simulink model "VHDModel"  (R2021b)
settings: Solver=VariableStepAuto  StartTime=0.0  StopTime=30  RelTol=1e-3
values from neighbouring files (symbols this model uses):
  CG_TO_FRONT_AXLE = 1.56    [VHD_parameters.m]
  CG_TO_REAR_AXLE = 1.04    [VHD_parameters.m]
  COEFICEINT_OF_FRICTION = 0.8    [VHD_parameters.m]
  FRONT_LATERAL_COEF = 14    [VHD_parameters.m]
  INERTIAL_MASS_MOMENT = 1360    [VHD_parameters.m]
  REAR_LATERAL_COEF = 13    [VHD_parameters.m]
  STEERING_RATIO = 1    [VHD_parameters.m]
  VEHICLE_MASS = 1600    [VHD_parameters.m]
  VEHICLE_TRACK = 1.7    [VHD_parameters.m]
  VELOCITY = 40    [VHD_parameters.m]
  WHEEL_BASE = 2.6    [VHD_parameters.m]
undefined symbols (not defined in the file or in its folder): magnitude
libraries: slpidlib x2, simulink_extras x2, simulink x1

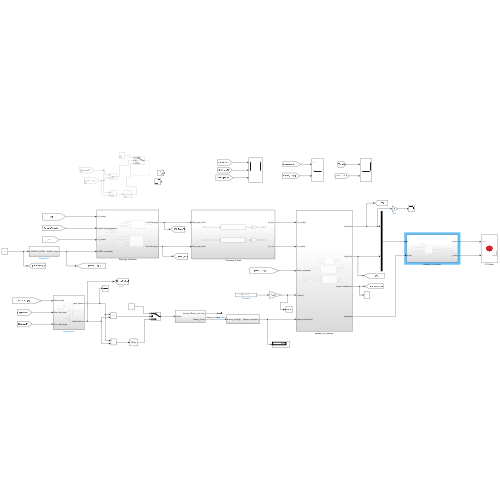
[thumbnail: Simulink's stored preview of the top-level diagram]
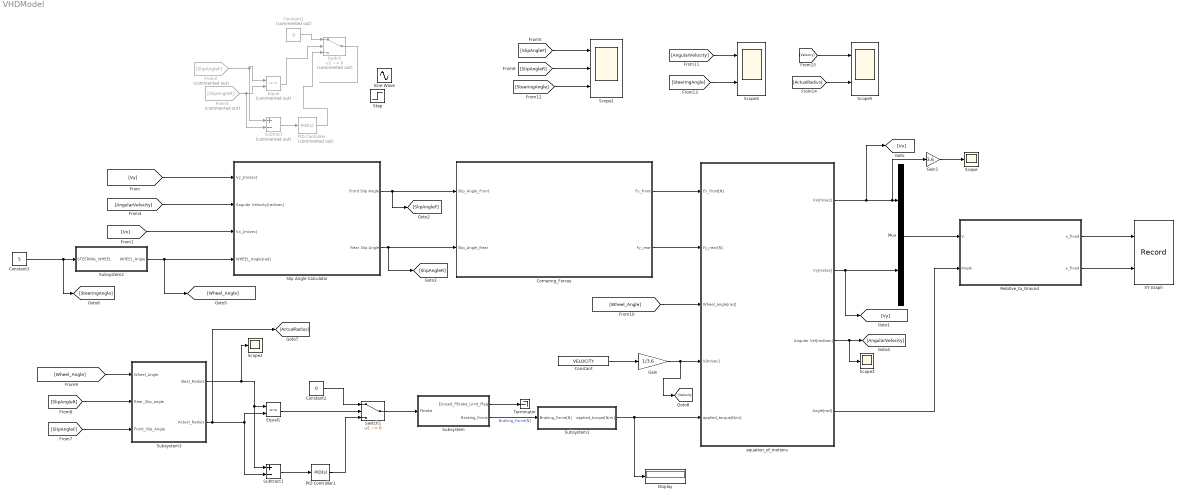
== system VHDModel ==
  Constant : Constant  Value=VELOCITY
  Constant1 : Constant  Commented=on  Value=0
  Constant2 : Constant  Value=0
  Constant3 : Constant  Value=5
  Cornering_Forces : Subsystem
  Display : Display
  Equal : RelationalOperator  Commented=on  Operator===  OutDataTypeStr=boolean  RndMeth=Simplest
  Equal1 : RelationalOperator  Operator===  OutDataTypeStr=boolean  RndMeth=Simplest
  From2 : From  Commented=on  GotoTag=SlipAngleF
  From3 : From  Commented=on  GotoTag=SlipAngleR
  Gain : Gain  Gain=1/3.6
  Gain1 : Gain  Gain=3.6
  Mux : Mux  Inputs=2
  PID Controller : slpidlib/PID Controller  Commented=on  Controller=PID  Form=Parallel  TimeDomain=Continuous-time  UseExternalTs=off  SampleTime=-1  IntegratorMethod=Forward Euler  FilterMethod=Forward Euler  ControllerParametersSource=internal  P=82.330505190178  I=12407.3336326962  D=0.077849176466117  UseFilter=on  N=20851.8597553552  TunerSelectOption=Transfer Function Based (PID Tuner App)  InitialConditionSource=internal  InitialConditionForIntegrator=0  InitialConditionForFilter=0  DifferentiatorICPrevScaledInput=0  ExternalReset=none  TrackingMode=off  Kt=1  LimitOutput=off  SatLimitsSource=internal  UpperSaturationLimit=inf  LowerSaturationLimit=-inf  LinearizeAsGain=on  AntiWindupMode=none  Kb=1  POutMin=[]  POutMax=[]  IOutMin=[]  IOutMax=[]  DOutMin=[]  DOutMax=[]  NOutMin=[]  NOutMax=[]  SumOutMin=[]  SumOutMax=[]  SaturationOutMin=[]  SaturationOutMax=[]  PParamMin=[]  PParamMax=[]  IParamMin=[]  IParamMax=[]  DParamMin=[]  DParamMax=[]  NParamMin=[]  NParamMax=[]  KbParamMin=[]  KbParamMax=[]  KtParamMin=[]  KtParamMax=[]  KbOutMin=[]  KbOutMax=[]  KtOutMin=[]  KtOutMax=[]  IntegratorOutMin=[]  IntegratorOutMax=[]  FilterOutMin=[]  FilterOutMax=[]  SumI1OutMin=[]  SumI1OutMax=[]  SumI2OutMin=[]  SumI2OutMax=[]  SumI3OutMin=[]  SumI3OutMax=[]  SumI4OutMin=[]  SumI4OutMax=[]  SumDOutMin=[]  SumDOutMax=[]  DifferentiatorOutMin=[]  DifferentiatorOutMax=[]  FilterDiffOutCoefMin=[]  FilterDiffOutCoefMax=[]  ReciprocalOutMin=[]  ReciprocalOutMax=[]  SumDenOutMin=[]  SumDenOutMax=[]  SumNumOutMin=[]  SumNumOutMax=[]  DivideOutMin=[]  DivideOutMax=[]  UdiffTsProdOutMin=[]  UdiffTsProdOutMax=[]  NTsProdOutMin=[]  NTsProdOutMax=[]  UintegralTsProdOutMin=[]  UintegralTsProdOutMax=[]  UngainTsProdOutMin=[]  UngainTsProdOutMax=[]  IntegratorContinuousStateAttributes=''  IntegratorStateMustResolveToSignalObject=off  IntegratorRTWStateStorageClass=Auto  FilterContinuousStateAttributes=''  FilterStateMustResolveToSignalObject=off  FilterRTWStateStorageClass=Auto  ParallelPVariant=InternalParameters  IdealPVariant=Disabled  IVariant=InternalParameters  DVariant=InternalParameters  IntegratorVariant=Continuous  SatVariant=Disabled  AWVariant=Passthrough  PCopyVariant=Disabled  TRVariant=Disabled  FdbkBlocksVariant=Forward  IdealPFdbkVariant=Disabled  SatFdbkVariant=Disabled  DerivativeFilterVariant=ContFilter  NVariant=InternalParameters  NCopyVariant=Disabled  FilterICVariant=InternalICsFilter  IntegratorICVariant=InternalICs  ExternalResetVariant=Disabled  TRSumVariant=Passthrough  SumFdbkVariant=Disabled  SumVariant=Sum_PID  TsampFilterVariant=InternalTs  TsampNgainVariant=Passthrough  TsampIntegralVariant=Passthrough  ExternalSaturationOutDataTypeStr=Inherit: Same as second input
  PID Controller1 : slpidlib/PID Controller  Controller=PID  Form=Parallel  TimeDomain=Continuous-time  UseExternalTs=off  SampleTime=-1  IntegratorMethod=Forward Euler  FilterMethod=Forward Euler  ControllerParametersSource=internal  P=-765.564265691975  I=-781534.171021295  D=-0.0269112999506061  UseFilter=on  N=5836.60149931409  TunerSelectOption=Transfer Function Based (PID Tuner App)  InitialConditionSource=internal  InitialConditionForIntegrator=0  InitialConditionForFilter=0  DifferentiatorICPrevScaledInput=0  ExternalReset=none  TrackingMode=off  Kt=1  LimitOutput=off  SatLimitsSource=internal  UpperSaturationLimit=inf  LowerSaturationLimit=-inf  LinearizeAsGain=on  AntiWindupMode=none  Kb=1  POutMin=[]  POutMax=[]  IOutMin=[]  IOutMax=[]  DOutMin=[]  DOutMax=[]  NOutMin=[]  NOutMax=[]  SumOutMin=[]  SumOutMax=[]  SaturationOutMin=[]  SaturationOutMax=[]  PParamMin=[]  PParamMax=[]  IParamMin=[]  IParamMax=[]  DParamMin=[]  DParamMax=[]  NParamMin=[]  NParamMax=[]  KbParamMin=[]  KbParamMax=[]  KtParamMin=[]  KtParamMax=[]  KbOutMin=[]  KbOutMax=[]  KtOutMin=[]  KtOutMax=[]  IntegratorOutMin=[]  IntegratorOutMax=[]  FilterOutMin=[]  FilterOutMax=[]  SumI1OutMin=[]  SumI1OutMax=[]  SumI2OutMin=[]  SumI2OutMax=[]  SumI3OutMin=[]  SumI3OutMax=[]  SumI4OutMin=[]  SumI4OutMax=[]  SumDOutMin=[]  SumDOutMax=[]  DifferentiatorOutMin=[]  DifferentiatorOutMax=[]  FilterDiffOutCoefMin=[]  FilterDiffOutCoefMax=[]  ReciprocalOutMin=[]  ReciprocalOutMax=[]  SumDenOutMin=[]  SumDenOutMax=[]  SumNumOutMin=[]  SumNumOutMax=[]  DivideOutMin=[]  DivideOutMax=[]  UdiffTsProdOutMin=[]  UdiffTsProdOutMax=[]  NTsProdOutMin=[]  NTsProdOutMax=[]  UintegralTsProdOutMin=[]  UintegralTsProdOutMax=[]  UngainTsProdOutMin=[]  UngainTsProdOutMax=[]  IntegratorContinuousStateAttributes=''  IntegratorStateMustResolveToSignalObject=off  IntegratorRTWStateStorageClass=Auto  FilterContinuousStateAttributes=''  FilterStateMustResolveToSignalObject=off  FilterRTWStateStorageClass=Auto  ParallelPVariant=InternalParameters  IdealPVariant=Disabled  IVariant=InternalParameters  DVariant=InternalParameters  IntegratorVariant=Continuous  SatVariant=Disabled  AWVariant=Passthrough  PCopyVariant=Disabled  TRVariant=Disabled  FdbkBlocksVariant=Forward  IdealPFdbkVariant=Disabled  SatFdbkVariant=Disabled  DerivativeFilterVariant=ContFilter  NVariant=InternalParameters  NCopyVariant=Disabled  FilterICVariant=InternalICsFilter  IntegratorICVariant=InternalICs  ExternalResetVariant=Disabled  TRSumVariant=Passthrough  SumFdbkVariant=Disabled  SumVariant=Sum_PID  TsampFilterVariant=InternalTs  TsampNgainVariant=Passthrough  TsampIntegralVariant=Passthrough  ExternalSaturationOutDataTypeStr=Inherit: Same as second input
  "Relative_to_Ground " : Subsystem
  Scope : Scope
  Scope1 : Scope  NumInputPorts=3
  Scope2 : Scope
  Scope3 : Scope
  Scope4 : Scope  NumInputPorts=2
  Scope5 : Scope  NumInputPorts=2
  Sine Wave : Sin  Amplitude=5  SampleTime=0
  Slip Angle Calculator : Subsystem
  Step : Step  After=5  SampleTime=0
  Subsystem : Subsystem
  Subsystem1 : Subsystem
  Subsystem2 : Subsystem
  Subsystem3 : Subsystem
  Subtract : Sum  Commented=on  Inputs=+-
  Subtract1 : Sum  Inputs=+-
  Switch : Switch  Commented=on  Criteria=u2 ~= 0
  Switch1 : Switch  Criteria=u2 ~= 0
  Terminator : Terminator
  XY Graph : Record  FileSettingsInternal="{\"entries\":[{\"content\":{\"excelSettings\":{\"content\":{},\"type\":\"Streamout.ExcelSettings\"}},\"type\":\"Streamout.FileSettingStorage\",\"uuid\":\"f7774bb4-364e-43f4-b193-5a8ab4c21426\"}],\"packageUris\":[\"http://schema.mathworks.com/mf0/streamout_blocks/R2020a\"],\"version\":\"1.0\"}"  Layout=[1 1]  SignalsInternal="{\"entries\":[{\"content\":{\"signals\":[{\"content\":{\"blockPath\":[\"untitled/XY Graph\"],\"channel\":[],\"dimensions\":[1],\"domain\":\"untitled/XY Graph\",\"lineColor\":\"#a2142f\",\"plots\":[1],\"port\":1,\"sid\":[\"\"],\"signalID\":8651,\"signalName\":\"Relative_to_Ground :1\"},\"type\":\"RecordBlkView.Signal\",\"uuid\":\"e4b58785-22ef-402e-9d41-1f1aedcd25fc\"},{\"content\":{\"blockPath\":[\"untitled/XY Graph\"],\"channel\":[],\"dimensions\":[1],\"domain\":\"untitled/XY Graph\",\"lineColor\":\"#139fff\",\"plots\":[1],\"port\":2,\"sid\":[\"\"],\"signalID\":8655,\"signalName\":\"Relative_to_Ground :2\"},\"type\":\"RecordBlkView.Signal\",\"uuid\":\"515ba19c-c257-45ec-a075-9a7a1776298c\"}]},\"type\":\"RecordBlkView.InputSignals\",\"uuid\":\"b163977e-3762-44b8-8902-6f00216ad88f\"}],\"packageUris\":[\"http://schema.mathworks.com/mf0/streamout_blocks/R2020a\"],\"version\":\"1.0\"}"  VisualizationBindings="{\"xyplotplugin\":{\"info\":[{\"series\":[{\"bindingParametersList\":[{\"parameter\":\"X-Axis\",\"signalID\":8651,\"signalName\":\"Relative_to_Ground :1\"},{\"parameter\":\"Y-Axis\",\"signalID\":8655,\"signalName\":\"Relative_to_Ground :2\"}],\"seriesID\":321}],\"subplotID\":1}]}}"  CompatibilityTag=XY  st=-1
  "equation_of_motions " : Subsystem
  wires:
  "equation_of_motions "/2(Vy[m/sec]) -> [Vy], Mux/2
  "equation_of_motions "/4(Angle[rad]) -> "Relative_to_Ground "/2(Angle)
  Equal/1 -> Switch/2
  Cornering_Forces/1(Fy_front) -> "equation_of_motions "/1(Fy_front[N])
  PID Controller/1 -> Switch/3
  Subtract/1 -> PID Controller/1
  Subsystem/1(Exceed_FBrake_Limit_Flag) -> Terminator/1
  [AngularVelocity] -> Slip Angle Calculator/2(Angular Velocity[rad/sec])
  [Wheel_Angle] -> Subsystem3/1(Wheel_Angle)
  Subsystem3/1(Ideal_Raduis) -> Scope2/1, Subtract1/1, Equal1/1
  [SlipAngleF] -> Subsystem3/3(Front_Slip_Angle)
  Subsystem2/1(WHEEL_Angle) -> [Wheel_Angle], Slip Angle Calculator/4(WHEEL_Angle[rad])
  [Vx] -> Slip Angle Calculator/3(Vx_[m/sec])
  "Relative_to_Ground "/1(x_fixed) -> XY Graph/1
  [ActualRadius] -> Scope5/2
  Slip Angle Calculator/2("Rear Slip Angle ") -> [SlipAngleR], Cornering_Forces/2(Slip_Angle_Rear)
  Constant1/1 -> Switch/1
  Constant3/1 -> [SteeringAngle], Subsystem2/1(STEERING_WHEEL)
  [Velocity] -> Scope5/1
  Constant2/1 -> Switch1/1
  [SteeringAngle] -> Scope4/2
  "Relative_to_Ground "/2(y_fixed) -> XY Graph/2
  Subsystem1/1(applied_torque[N/m]) -> Display/1, "equation_of_motions "/5(applied_torque[N/m])
  [Vy] -> Slip Angle Calculator/1(Vy_[m/sec])
  Gain/1 -> [Velocity], "equation_of_motions "/4(V[m/sec])
  Subtract1/1 -> PID Controller1/1
  "equation_of_motions "/1(Vx[m/sec]) -> [Vx], Gain1/1, Mux/1
  [AngularVelocity] -> Scope4/1
  [Wheel_Angle] -> "equation_of_motions "/3(Wheel_angle[rad])
  Gain1/1 -> Scope/1
  PID Controller1/1 -> Switch1/3
  [SlipAngleF] -> Scope1/1
  Constant/1 -> Gain/1
  Subsystem3/2(Actual_Raduis) -> [ActualRadius], Subtract1/2, Equal1/2
  Equal1/1 -> Switch1/2
  [SlipAngleR] -> Scope1/2
  [SlipAngleR] -> Subsystem3/2(Rear_Slip_angle)
  [SteeringAngle] -> Scope1/3
  "equation_of_motions "/3(Angular Vel[rad/sec]) -> Scope3/1, [AngularVelocity]
  Switch1/1 -> Subsystem/1(Fbrake)
  From3/1 -> Subtract/2, Equal/2
  Mux/1 -> "Relative_to_Ground "/1(V)
  From2/1 -> Equal/1, Subtract/1
  Cornering_Forces/2(Fy_rear) -> "equation_of_motions "/2(Fy_rear[N])
  Subsystem/2(Braking_Force) -> Subsystem1/1(Braking_Force[N])  "Braking_Force[N]"
  Slip Angle Calculator/1(Front Slip Angle) -> Cornering_Forces/1(Slip_Angle_Front), [SlipAngleF]
  Switch/1 -> ?

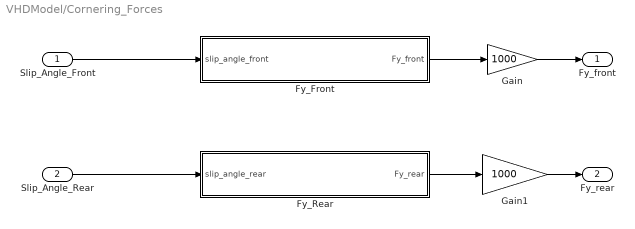
== system VHDModel/Cornering_Forces ==
  Slip_Angle_Front : Inport
  Slip_Angle_Rear : Inport  Port=2
  Fy_Front : Subsystem
  Fy_Rear : Subsystem
  Gain : Gain  Gain=1000
  Gain1 : Gain  Gain=1000
  Fy_front : Outport  VectorParamsAs1DForOutWhenUnconnected=off
  Fy_rear : Outport  Port=2  VectorParamsAs1DForOutWhenUnconnected=off
  wires:
  Fy_Rear/1(Fy_rear) -> Gain1/1
  Fy_Front/1(Fy_front) -> Gain/1
  Slip_Angle_Rear/1 -> Fy_Rear/1(slip_angle_rear)
  Slip_Angle_Front/1 -> Fy_Front/1(slip_angle_front)
  Gain/1 -> Fy_front/1
  Gain1/1 -> Fy_rear/1

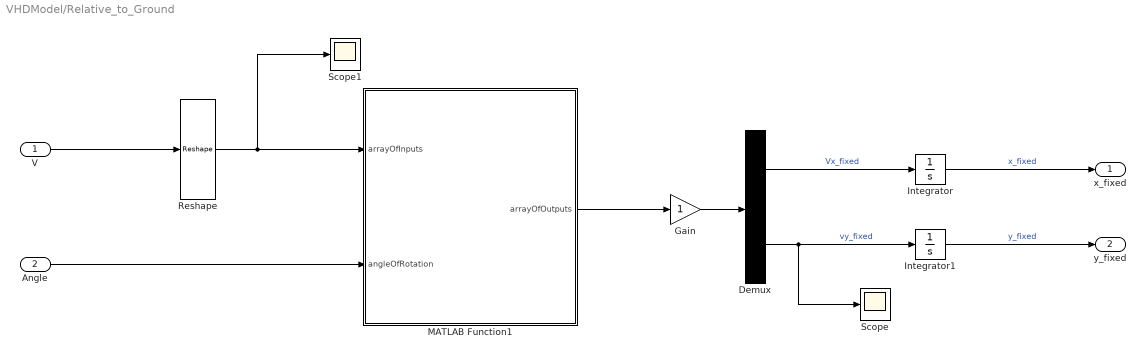
== system VHDModel/Relative_to_Ground  ==
  V : Inport
  Angle : Inport  Port=2
  Demux : Demux  Outputs=2
  Gain : Gain
  Integrator : Integrator
  Integrator1 : Integrator
  MATLAB Function1 : MATLAB Function  TreatAsAtomicUnit=on
  Reshape : Reshape  OutputDimensionality=Column vector (2-D)
  Scope : Scope
  Scope1 : Scope
  x_fixed : Outport  VectorParamsAs1DForOutWhenUnconnected=off
  y_fixed : Outport  Port=2  VectorParamsAs1DForOutWhenUnconnected=off
  wires:
  Demux/1 -> Integrator/1  "Vx_fixed"
  Angle/1 -> MATLAB Function1/2(angleOfRotation)
  Demux/2 -> Scope/1, Integrator1/1  "vy_fixed"
  Gain/1 -> Demux/1
  Reshape/1 -> Scope1/1, MATLAB Function1/1(arrayOfInputs)
  Integrator1/1 -> y_fixed/1  "y_fixed"
  V/1 -> Reshape/1
  MATLAB Function1/1(arrayOfOutputs) -> Gain/1
  Integrator/1 -> x_fixed/1  "x_fixed"

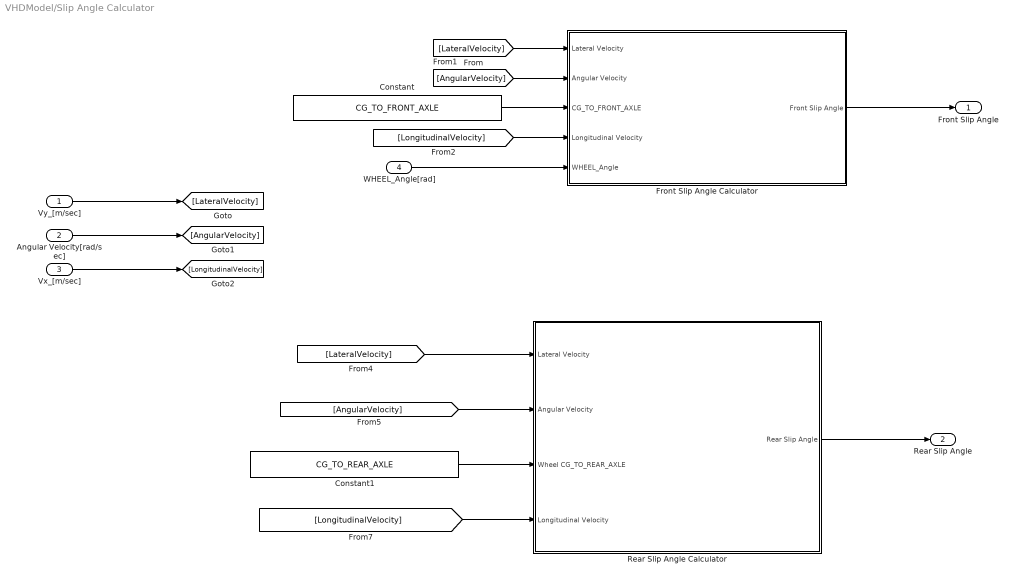
== system VHDModel/Slip Angle Calculator ==
  Vy_[m/sec] : Inport
  Angular Velocity[rad/sec] : Inport  Port=2
  Vx_[m/sec] : Inport  Port=3
  WHEEL_Angle[rad] : Inport  Port=4
  Constant : Constant  Value=CG_TO_FRONT_AXLE
  Constant1 : Constant  Value=CG_TO_REAR_AXLE
  Front Slip Angle Calculator : Subsystem
  Rear Slip Angle Calculator : Subsystem
  Front Slip Angle : Outport
  "Rear Slip Angle " : Outport  Port=2
  wires:
  [AngularVelocity] -> Front Slip Angle Calculator/2(Angular Velocity)
  WHEEL_Angle[rad]/1 -> Front Slip Angle Calculator/5(WHEEL_Angle)
  [LateralVelocity] -> Front Slip Angle Calculator/1(Lateral Velocity)
  Angular Velocity[rad/sec]/1 -> [AngularVelocity]
  Vx_[m/sec]/1 -> [LongitudinalVelocity]
  [LateralVelocity] -> Rear Slip Angle Calculator/1(Lateral Velocity)
  [LongitudinalVelocity] -> Front Slip Angle Calculator/4(Longitudinal Velocity)
  [AngularVelocity] -> Rear Slip Angle Calculator/2(Angular Velocity)
  [LongitudinalVelocity] -> Rear Slip Angle Calculator/4(Longitudinal Velocity)
  Vy_[m/sec]/1 -> [LateralVelocity]
  Rear Slip Angle Calculator/1("Rear Slip Angle ") -> "Rear Slip Angle "/1
  Constant/1 -> Front Slip Angle Calculator/3(CG_TO_FRONT_AXLE)
  Front Slip Angle Calculator/1(Front Slip Angle) -> Front Slip Angle/1
  Constant1/1 -> Rear Slip Angle Calculator/3(Wheel CG_TO_REAR_AXLE)

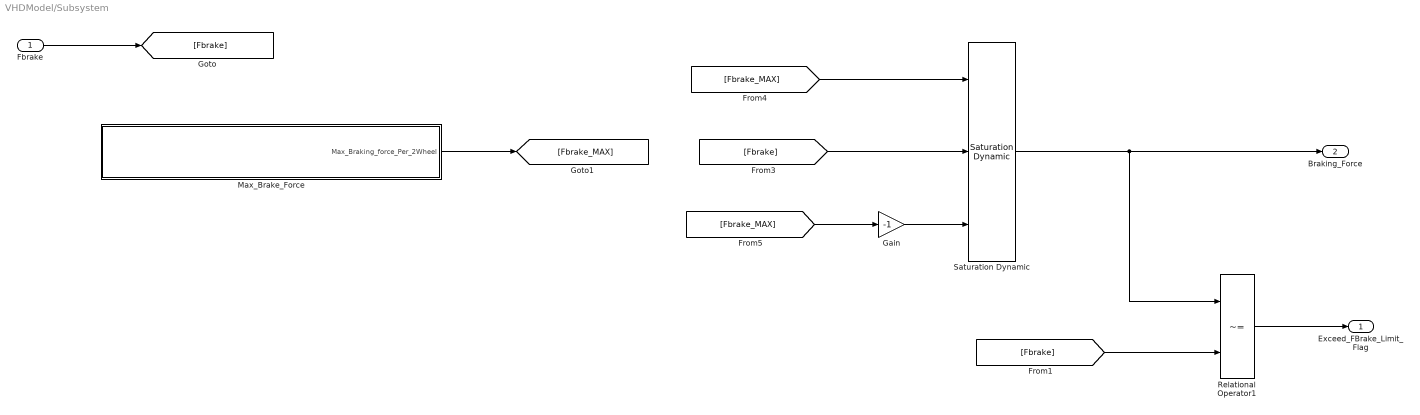
== system VHDModel/Subsystem ==
  Fbrake : Inport
  Gain : Gain  Gain=-1
  Max_Brake_Force : Subsystem
  Relational Operator1 : RelationalOperator  Operator=~=  OutDataTypeStr=boolean  RndMeth=Simplest
  Saturation Dynamic : simulink/Discontinuities/Saturation Dynamic  OutMin=[]  OutMax=[]  OutDataTypeStr=Inherit: Same as second input  OutDataType=fixdt(1, 16)  OutScaling=2^-10  DoSatur=off
  Exceed_FBrake_Limit_Flag : Outport  VectorParamsAs1DForOutWhenUnconnected=off
  Braking_Force : Outport  Port=2  VectorParamsAs1DForOutWhenUnconnected=off
  wires:
  Fbrake/1 -> [Fbrake]
  Max_Brake_Force/1(Max_Braking_force_Per_2Wheel) -> [Fbrake_MAX]
  [Fbrake] -> Saturation Dynamic/2
  [Fbrake_MAX] -> Saturation Dynamic/1
  [Fbrake_MAX] -> Gain/1
  Gain/1 -> Saturation Dynamic/3
  Saturation Dynamic/1 -> Relational Operator1/1, Braking_Force/1
  [Fbrake] -> Relational Operator1/2
  Relational Operator1/1 -> Exceed_FBrake_Limit_Flag/1

== system VHDModel/Subsystem1 ==
  Braking_Force[N] : Inport
  Constant : Constant  Value=VEHICLE_TRACK
  Gain : Gain  Gain=1/2
  Product : Product
  applied_torque[N/m] : Outport  VectorParamsAs1DForOutWhenUnconnected=off
  wires:
  Gain/1 -> Product/2
  Product/1 -> applied_torque[N/m]/1  "applied_torque"
  Constant/1 -> Gain/1  "vehicle_track[m]"
  Braking_Force[N]/1 -> Product/1

== system VHDModel/Subsystem2 ==
  STEERING_WHEEL : Inport
  Constant : Constant  Value=STEERING_RATIO
  Degrees to Radians : simulink_extras/Transformations/Degrees to Radians
  Product : Product
  Saturation : Saturate  UpperLimit=40  LowerLimit=-40
  WHEEL_Angle : Outport  VectorParamsAs1DForOutWhenUnconnected=off
  wires:
  Product/1 -> Saturation/1  "WHEEL_Angle[deg]"
  STEERING_WHEEL/1 -> Product/1
  Degrees to Radians/1 -> WHEEL_Angle/1  "WHEEL_Angle[rad]"
  Constant/1 -> Product/2
  Saturation/1 -> Degrees to Radians/1

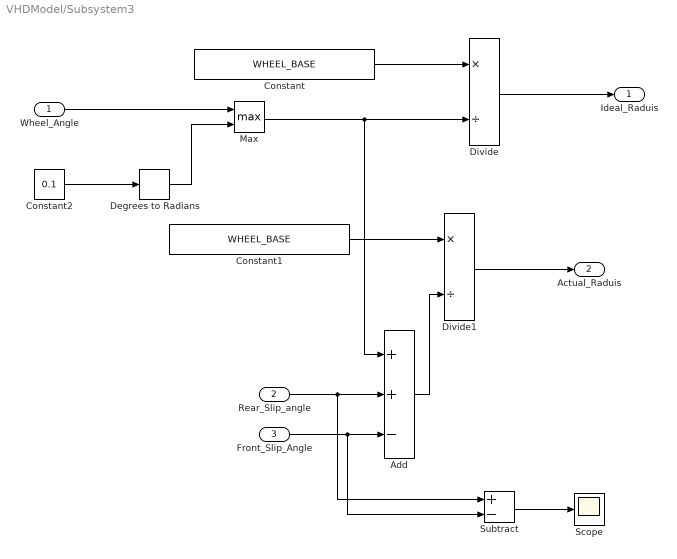
== system VHDModel/Subsystem3 ==
  Wheel_Angle : Inport
  Rear_Slip_angle : Inport  Port=2
  Front_Slip_Angle : Inport  Port=3
  Add : Sum  Inputs=++-
  Constant : Constant  Value=WHEEL_BASE
  Constant1 : Constant  Value=WHEEL_BASE
  Constant2 : Constant  Value=0.1
  Degrees to Radians : simulink_extras/Transformations/Degrees to Radians
  Divide : Product  Inputs=*/  OutDataTypeStr=Inherit: Inherit via back propagation
  Divide1 : Product  Inputs=*/  OutDataTypeStr=Inherit: Inherit via back propagation
  Max : MinMax  Function=max  Inputs=2
  Scope : Scope
  Subtract : Sum  Inputs=+-
  Ideal_Raduis : Outport  VectorParamsAs1DForOutWhenUnconnected=off
  Actual_Raduis : Outport  Port=2  VectorParamsAs1DForOutWhenUnconnected=off
  wires:
  Wheel_Angle/1 -> Max/1
  Constant/1 -> Divide/1
  Constant1/1 -> Divide1/1
  Rear_Slip_angle/1 -> Subtract/1, Add/2
  Front_Slip_Angle/1 -> Subtract/2, Add/3
  Add/1 -> Divide1/2
  Divide1/1 -> Actual_Raduis/1
  Subtract/1 -> Scope/1
  Max/1 -> Add/1, Divide/2
  Constant2/1 -> Degrees to Radians/1
  Divide/1 -> Ideal_Raduis/1
  Degrees to Radians/1 -> Max/2

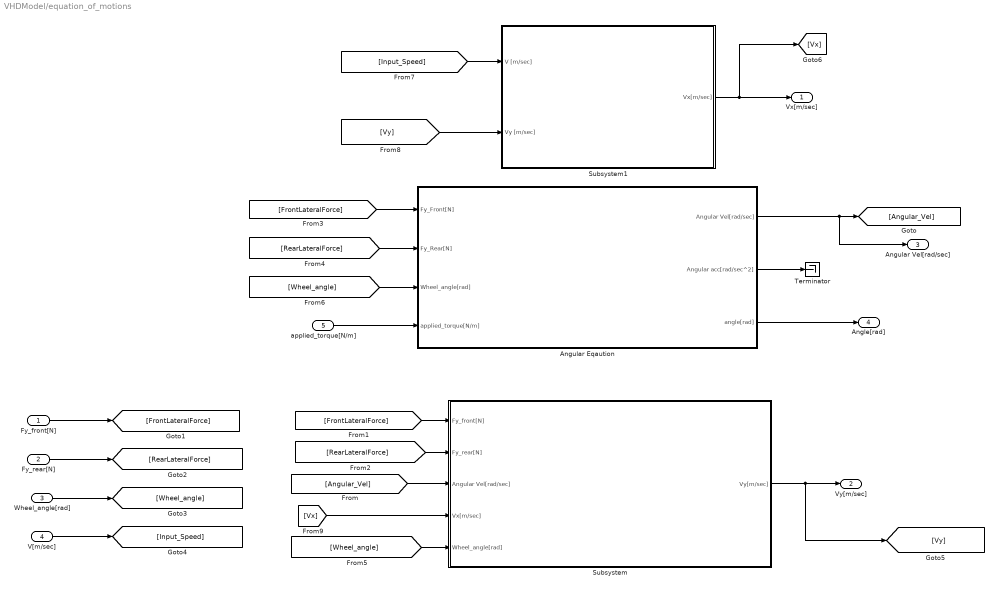
== system VHDModel/equation_of_motions  ==
  Fy_front[N] : Inport
  Fy_rear[N] : Inport  Port=2
  Wheel_angle[rad] : Inport  Port=3
  V[m/sec] : Inport  Port=4
  applied_torque[N/m] : Inport  Port=5
  "Angular Eqaution " : Subsystem
  Subsystem : Subsystem
  Subsystem1 : Subsystem
  Terminator : Terminator
  Vx[m/sec] : Outport  VectorParamsAs1DForOutWhenUnconnected=off
  Vy[m/sec] : Outport  Port=2  VectorParamsAs1DForOutWhenUnconnected=off
  Angular Vel[rad/sec] : Outport  Port=3  VectorParamsAs1DForOutWhenUnconnected=off
  Angle[rad] : Outport  Port=4  VectorParamsAs1DForOutWhenUnconnected=off
  wires:
  "Angular Eqaution "/1(Angular Vel[rad/sec]) -> Angular Vel[rad/sec]/1, [Angular_Vel]
  [Angular_Vel] -> Subsystem/3(Angular Vel[rad/sec])
  "Angular Eqaution "/2(Angular acc[rad/sec^2]) -> Terminator/1
  "Angular Eqaution "/3(angle[rad]) -> Angle[rad]/1
  Fy_front[N]/1 -> [FrontLateralForce]
  Fy_rear[N]/1 -> [RearLateralForce]
  [FrontLateralForce] -> Subsystem/1(Fy_front[N])
  [RearLateralForce] -> Subsystem/2(Fy_rear[N])
  [FrontLateralForce] -> "Angular Eqaution "/1(Fy_Front[N])
  [RearLateralForce] -> "Angular Eqaution "/2(Fy_Rear[N])
  Wheel_angle[rad]/1 -> [Wheel_angle]
  [Wheel_angle] -> Subsystem/5(Wheel_angle[rad])
  [Wheel_angle] -> "Angular Eqaution "/3(Wheel_angle[rad])
  applied_torque[N/m]/1 -> "Angular Eqaution "/4(applied_torque[N/m])
  V[m/sec]/1 -> [Input_Speed]
  Subsystem/1(Vy[m/sec]) -> [Vy], Vy[m/sec]/1
  Subsystem1/1(Vx[m/sec]) -> [Vx], Vx[m/sec]/1
  [Input_Speed] -> Subsystem1/1(V [m/sec])
  [Vx] -> Subsystem/4(Vx[m/sec])
  [Vy] -> Subsystem1/2(Vy [m/sec])

== system VHDModel/Cornering_Forces/Fy_Front ==
  slip_angle_front : Inport
  Constant : Constant  Value=FRONT_LATERAL_COEF
  Constant1 : Constant  Value=2
  Product : Product
  Product1 : Product
  Fy_front : Outport  VectorParamsAs1DForOutWhenUnconnected=off
  wires:
  slip_angle_front/1 -> Product/1
  Constant/1 -> Product/2
  Product/1 -> Product1/1
  Constant1/1 -> Product1/2
  Product1/1 -> Fy_front/1

== system VHDModel/Cornering_Forces/Fy_Rear ==
  slip_angle_rear : Inport
  Constant : Constant  Value=REAR_LATERAL_COEF
  Constant1 : Constant  Value=2
  Product : Product
  Product1 : Product
  Fy_rear : Outport  VectorParamsAs1DForOutWhenUnconnected=off
  wires:
  Product1/1 -> Fy_rear/1
  Constant1/1 -> Product1/2
  Product/1 -> Product1/1
  Constant/1 -> Product/2
  slip_angle_rear/1 -> Product/1

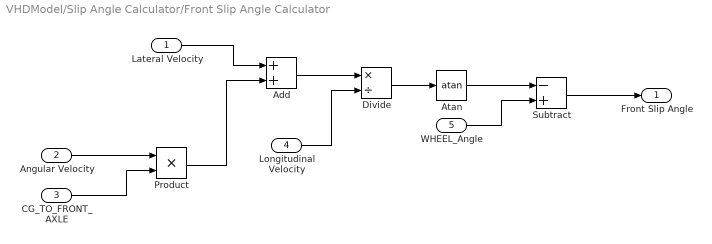
== system VHDModel/Slip Angle Calculator/Front Slip Angle Calculator ==
  Lateral Velocity : Inport
  Angular Velocity : Inport  Port=2
  CG_TO_FRONT_AXLE : Inport  Port=3
  Longitudinal Velocity : Inport  Port=4
  WHEEL_Angle : Inport  Port=5
  Add : Sum
  Atan : Trigonometry  Operator=atan
  Divide : Product  Inputs=*/
  Product : Product
  Subtract : Sum  Inputs=-+
  Front Slip Angle : Outport
  wires:
  Add/1 -> Divide/1
  Product/1 -> Add/2
  CG_TO_FRONT_AXLE/1 -> Product/2
  Lateral Velocity/1 -> Add/1
  WHEEL_Angle/1 -> Subtract/2
  Subtract/1 -> Front Slip Angle/1
  Longitudinal Velocity/1 -> Divide/2
  Angular Velocity/1 -> Product/1
  Divide/1 -> Atan/1
  Atan/1 -> Subtract/1

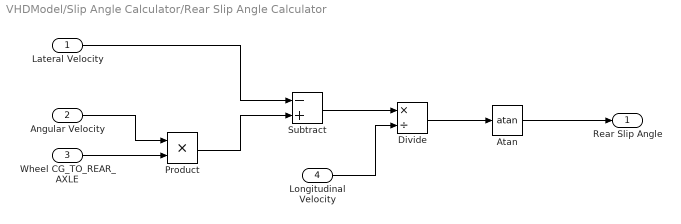
== system VHDModel/Slip Angle Calculator/Rear Slip Angle Calculator ==
  Lateral Velocity : Inport
  Angular Velocity : Inport  Port=2
  Wheel CG_TO_REAR_AXLE : Inport  Port=3
  Longitudinal Velocity : Inport  Port=4
  Atan : Trigonometry  Operator=atan
  Divide : Product  Inputs=*/
  Product : Product
  Subtract : Sum  Inputs=-+
  "Rear Slip Angle " : Outport
  wires:
  Angular Velocity/1 -> Product/1
  Product/1 -> Subtract/2
  Longitudinal Velocity/1 -> Divide/2
  Lateral Velocity/1 -> Subtract/1
  Wheel CG_TO_REAR_AXLE/1 -> Product/2
  Subtract/1 -> Divide/1
  Divide/1 -> Atan/1
  Atan/1 -> "Rear Slip Angle "/1

== system VHDModel/Subsystem/Max_Brake_Force ==
  Constant : Constant  Value=VEHICLE_MASS
  Constant1 : Constant  Value=9.81
  Constant2 : Constant  Value=COEFICEINT_OF_FRICTION
  Gain : Gain  Gain=1/2
  Product : Product  Inputs=3
  Max_Braking_force_Per_2Wheel : Outport  VectorParamsAs1DForOutWhenUnconnected=off
  wires:
  Constant/1 -> Product/1
  Product/1 -> Gain/1  "total_Max_Braking_force"
  Constant2/1 -> Product/3
  Constant1/1 -> Product/2  "gravitational_acc"
  Gain/1 -> Max_Braking_force_Per_2Wheel/1  "Max_Braking_force_Per_2Wheel"

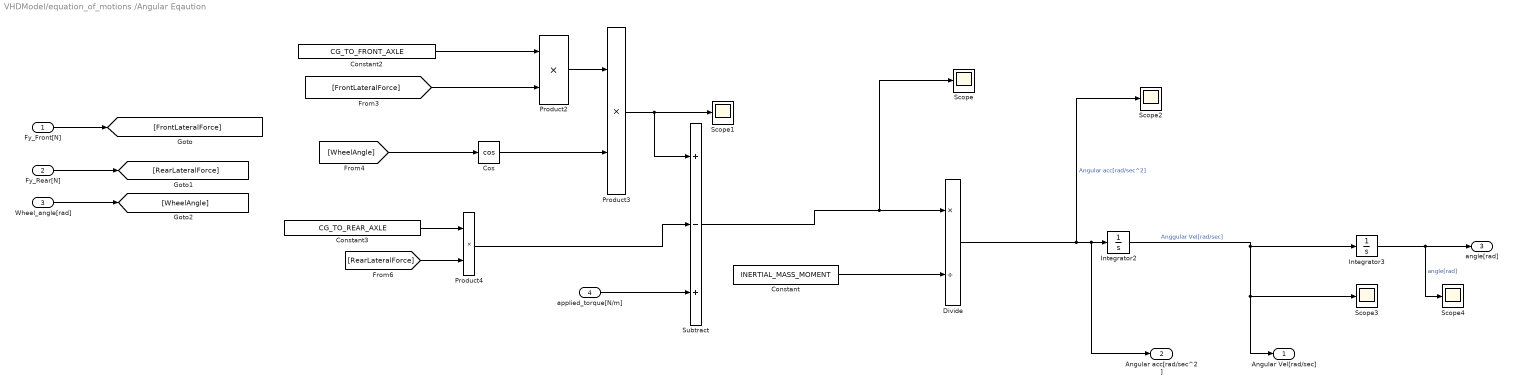
== system VHDModel/equation_of_motions /Angular Eqaution  ==
  Fy_Front[N] : Inport
  Fy_Rear[N] : Inport  Port=2
  Wheel_angle[rad] : Inport  Port=3
  applied_torque[N/m] : Inport  Port=4
  Constant : Constant  Value=INERTIAL_MASS_MOMENT
  Constant2 : Constant  Value=CG_TO_FRONT_AXLE
  Constant3 : Constant  Value=CG_TO_REAR_AXLE
  Cos : Trigonometry  Operator=cos
  Divide : Product  Inputs=*/  OutDataTypeStr=Inherit: Inherit via back propagation
  Integrator2 : Integrator  InitialCondition=0.01
  Integrator3 : Integrator
  Product2 : Product
  Product3 : Product
  Product4 : Product
  Scope{,1..4} (5 alike) : Scope
  Subtract : Sum  Inputs=+-+
  Angular Vel[rad/sec] : Outport  VectorParamsAs1DForOutWhenUnconnected=off
  Angular acc[rad/sec^2] : Outport  Port=2  VectorParamsAs1DForOutWhenUnconnected=off
  angle[rad] : Outport  Port=3  VectorParamsAs1DForOutWhenUnconnected=off
  wires:
  Product3/1 -> Scope1/1, Subtract/1
  [WheelAngle] -> Cos/1
  Divide/1 -> Scope2/1, Integrator2/1, Angular acc[rad/sec^2]/1  "Angular acc[rad/sec^2]"
  [RearLateralForce] -> Product4/2
  Integrator2/1 -> Angular Vel[rad/sec]/1, Scope3/1, Integrator3/1  "Anggular Vel[rad/sec]"
  Subtract/1 -> Scope/1, Divide/1
  Product4/1 -> Subtract/2
  Integrator3/1 -> angle[rad]/1, Scope4/1  "angle[rad]"
  Constant2/1 -> Product2/1
  Constant3/1 -> Product4/1
  Product2/1 -> Product3/1
  [FrontLateralForce] -> Product2/2
  Fy_Front[N]/1 -> [FrontLateralForce]
  Fy_Rear[N]/1 -> [RearLateralForce]
  Wheel_angle[rad]/1 -> [WheelAngle]
  Cos/1 -> Product3/2
  applied_torque[N/m]/1 -> Subtract/3
  Constant/1 -> Divide/2

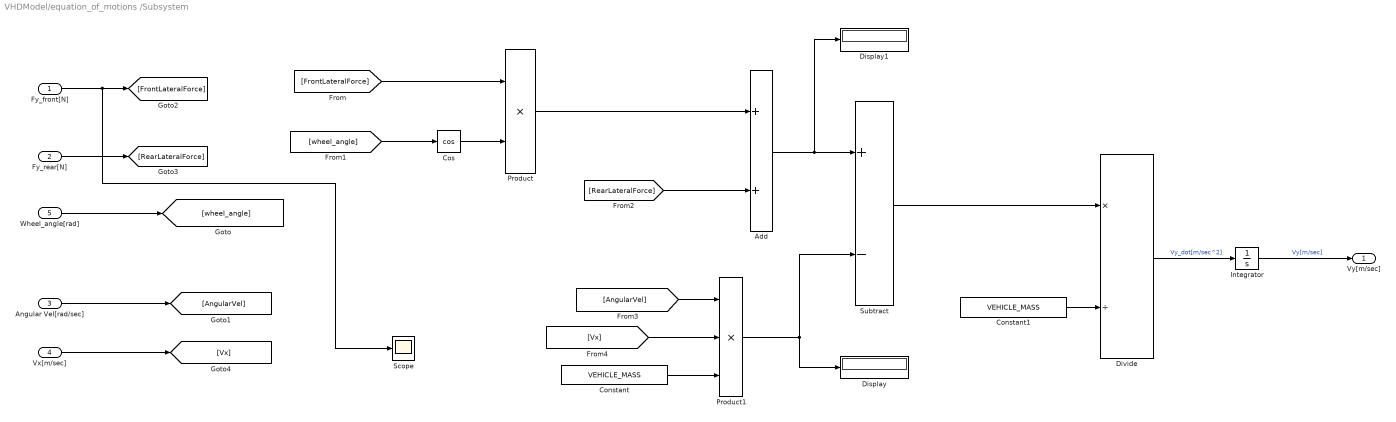
== system VHDModel/equation_of_motions /Subsystem ==
  Fy_front[N] : Inport
  Fy_rear[N] : Inport  Port=2
  Angular Vel[rad/sec] : Inport  Port=3
  Vx[m/sec] : Inport  Port=4
  Wheel_angle[rad] : Inport  Port=5
  Add : Sum
  Constant : Constant  Value=VEHICLE_MASS
  Constant1 : Constant  Value=VEHICLE_MASS
  Cos : Trigonometry  Operator=cos
  Display : Display
  Display1 : Display
  Divide : Product  Inputs=*/
  Integrator : Integrator
  Product : Product
  Product1 : Product  Inputs=3
  Scope : Scope
  Subtract : Sum  Inputs=+-
  Vy[m/sec] : Outport  VectorParamsAs1DForOutWhenUnconnected=off
  wires:
  Constant/1 -> Product1/3
  Vx[m/sec]/1 -> [Vx]
  Fy_rear[N]/1 -> [RearLateralForce]
  Product/1 -> Add/1
  [wheel_angle] -> Cos/1
  Cos/1 -> Product/2
  Subtract/1 -> Divide/1
  [Vx] -> Product1/2
  Product1/1 -> Subtract/2, Display/1
  [RearLateralForce] -> Add/2
  Fy_front[N]/1 -> Scope/1, [FrontLateralForce]
  Integrator/1 -> Vy[m/sec]/1  "Vy[m/sec]"
  Divide/1 -> Integrator/1  "Vy_dot[m/sec^2]"
  Angular Vel[rad/sec]/1 -> [AngularVel]
  [AngularVel] -> Product1/1
  Add/1 -> Display1/1, Subtract/1
  [FrontLateralForce] -> Product/1
  Constant1/1 -> Divide/2
  Wheel_angle[rad]/1 -> [wheel_angle]

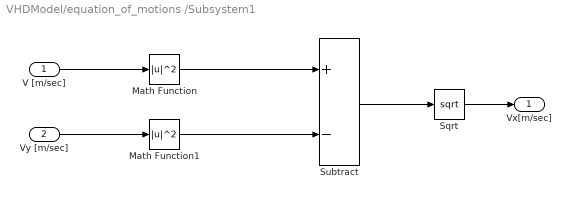
== system VHDModel/equation_of_motions /Subsystem1 ==
  V [m/sec] : Inport
  Vy [m/sec] : Inport  Port=2
  Math Function : Math  Operator=magnitude^2  SignedPower=on  SaturateOnIntegerOverflow=on
  Math Function1 : Math  Operator=magnitude^2  SignedPower=on  SaturateOnIntegerOverflow=on
  Sqrt : Sqrt  SaturateOnIntegerOverflow=on
  Subtract : Sum  Inputs=+-
  Vx[m/sec] : Outport  VectorParamsAs1DForOutWhenUnconnected=off
  wires:
  V [m/sec]/1 -> Math Function/1
  Sqrt/1 -> Vx[m/sec]/1
  Vy [m/sec]/1 -> Math Function1/1
  Subtract/1 -> Sqrt/1
  Math Function/1 -> Subtract/1
  Math Function1/1 -> Subtract/2

== matlab function VHDModel/Relative_to_Ground /MATLAB Function1 ==
  data: arrayOfInputs input; arrayOfOutputs output; angleOfRotation input
function arrayOfOutputs = fcn(arrayOfInputs, angleOfRotation)
tf = [cos(angleOfRotation) -sin(angleOfRotation);sin(angleOfRotation) cos(angleOfRotation)];
arrayOfOutputs = inv(tf)*arrayOfInputs;
